simulink subsystem "Sonars"  (R2022b)
settings: Solver=VariableStepAuto  StartTime=0.0  StopTime=10.0  RelTol=1e-3
libraries: arduinolib x2
settings Model: Creator=miriamfreiriasanjuan  LastModifiedBy=miriamfreiriasanjuan

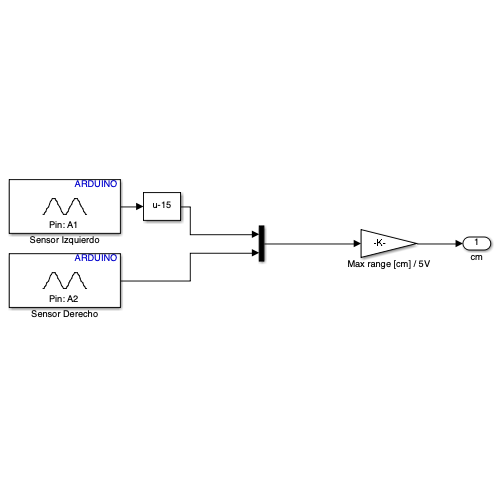
[thumbnail: Simulink's stored preview of the top-level diagram]
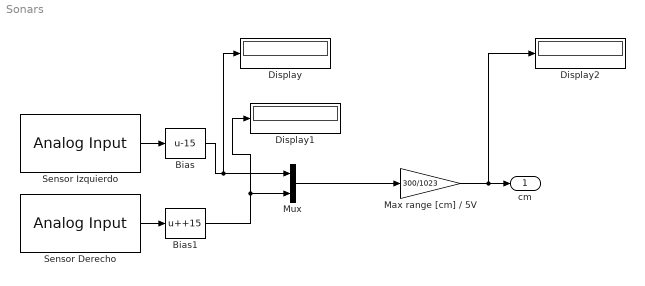
== system Sonars ==
  Bias : Bias  Bias=-15  SaturateOnIntegerOverflow=off
  Bias1 : Bias  Bias=+15  SaturateOnIntegerOverflow=off
  Display : Display
  Display1 : Display
  Display2 : Display
  Max range [cm] / 5V : Gain  Gain=300/1023
  Mux : Mux  Inputs=2
  Sensor Derecho : arduinolib/Analog Input  pinNumber=2  ReadResultsOnly=off  ConversionTriggerSource=Software  ExternalTriggerType=uint32( 0 )  OutputDataType=uint16  EnableConversionCompleteNotify=off  EnableOuputStatus=off  SampleTime=0.1  blockPlatform=arduino
  Sensor Izquierdo : arduinolib/Analog Input  pinNumber=1  ReadResultsOnly=off  ConversionTriggerSource=Software  ExternalTriggerType=uint32( 0 )  OutputDataType=uint16  EnableConversionCompleteNotify=off  EnableOuputStatus=off  SampleTime=0.1  blockPlatform=arduino
  cm : Outport
  wires:
  Sensor Derecho/1 -> Bias1/1
  Bias/1 -> Display/1, Mux/1
  Sensor Izquierdo/1 -> Bias/1
  Mux/1 -> Max range [cm] / 5V/1
  Max range [cm] / 5V/1 -> cm/1, Display2/1
  Bias1/1 -> Mux/2, Display1/1
